simulink model "lab2"  (R2024a)
settings: Solver=VariableStepAuto  StartTime=0.0  StopTime=10.0  RelTol=1e-3
settings Model: Creator=nikitza  LastModifiedBy=nikitza

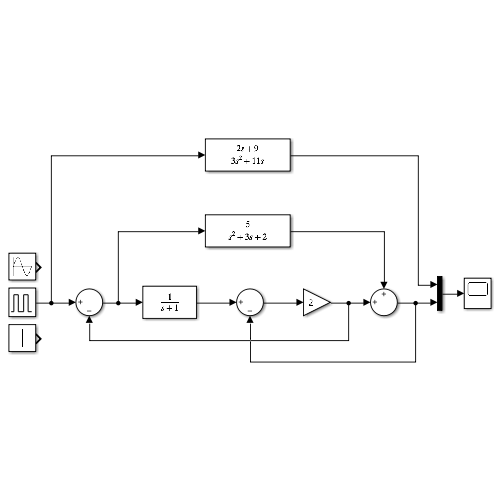
[thumbnail: Simulink's stored preview of the top-level diagram]
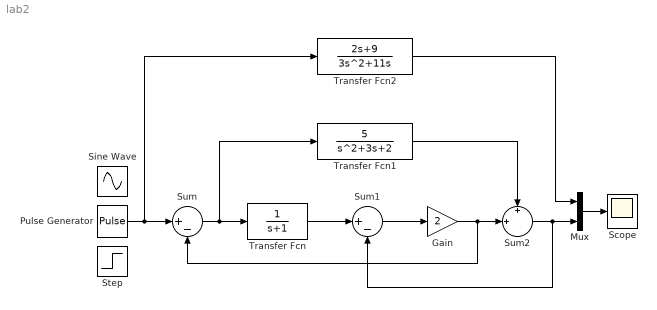
== system lab2 ==
  Gain : Gain  Gain=2
  Mux : Mux  Inputs=2
  Pulse Generator : DiscretePulseGenerator  PulseType=Time based  Period=10  PulseWidth=5
  Scope : Scope
  Sine Wave : Sin  SampleTime=0
  Step : Step  SampleTime=0
  Sum : Sum  Inputs=|+-
  Sum1 : Sum  Inputs=|+-
  Sum2 : Sum  Inputs=+|+||
  Transfer Fcn : TransferFcn  Denominator=[1 1]
  Transfer Fcn1 : TransferFcn  Numerator=[5]  Denominator=[1 3 2]
  Transfer Fcn2 : TransferFcn  Numerator=[2 9]  Denominator=[3 11 0]
  wires:
  Pulse Generator/1 -> Sum/1, Transfer Fcn2/1
  Sum/1 -> Transfer Fcn1/1, Transfer Fcn/1
  Transfer Fcn/1 -> Sum1/1
  Sum1/1 -> Gain/1
  Transfer Fcn1/1 -> Sum2/1
  Gain/1 -> Sum/2, Sum2/2
  Sum2/1 -> Sum1/2, Mux/2
  Transfer Fcn2/1 -> Mux/1
  Mux/1 -> Scope/1
